simulink model "VehicleSignals"  (R2024a)
settings: Solver=FixedStepDiscrete  StartTime=0.0  StopTime=VSG_Stop_Time  FixedStep=VSG_Step_Size  RelTol=1e-3  EnableMultiTasking=on
undefined symbols (not defined in the file): GEAR_FAILSAFE, Gear_T, RadarStatus_T, SignalStatus_T, STEER_FAILSAFE_DEG, STEER_RAW_MAX, STEER_RAW_MIN, STEER_RESOLUTION_DEG, TurnSignal_T, VSG_RECOVERY_CNT, VSPD_FAILSAFE_KMH, VSPD_RAW_MAX, VSPD_RAW_MIN, VSPD_RESOLUTION_KMH
libraries: simulink x10
settings Model: DataDictionary=bsd.sldd  Creator=pc  LastModifiedBy=pc
settings OptimizationCC: DefaultParameterBehavior=Inlined  UseDivisionForNetSlopeComputation=on  DefaultUnderspecifiedDataType=single  EnhancedBackFolding=on  PassReuseOutputArgsAs=Individual arguments  ZeroExternalMemoryAtStartup=off  ZeroInternalMemoryAtStartup=off  OptimizeBlockOrder=speed  DifferentSizesBufferReuse=on  OptimizationCustomize=off  EfficientTunableParamExpr=on
settings DebuggingCC: ParameterTunabilityLossMsg=error
settings SFSimCC: MATLABDynamicMemAlloc=off
settings RTWCC: Description=AUTOSAR  SystemTargetFile=autosar.tlc  GenCodeOnly=on  TemplateMakefile=ert_default_tmf  DataTypeReplacement=CDataTypesFixedWidth
settings CodeAppCC: ForceParamTrailComments=on  IgnoreCustomStorageClasses=off  OperatorAnnotations=on  SimulinkDataObjDesc=on  SFDataObjDesc=on  InsertBlockDesc=on
settings STFCustomTargetCC: MultiwordLength=256  ParMdlRefBuildCompliant=on  CompOptLevelCompliant=on  IncludeMdlTerminateFcn=off  CombineOutputUpdateFcns=on  SuppressErrorStatus=on  ERTCustomFileBanners=on  SupportNonFinite=off  SupportComplex=off  SupportContinuousTime=off  SupportNonInlinedSFcns=off  RemoveResetFunc=on  MATLABClassNameForMDSCustomization=Simulink.SoftwareTarget.ERTCustomization  AutosarCompliant=on  GRTInterface=off  LookupTableObjectStructAxisOrder=2,1,3,4,...  LUTObjectStructOrderEvenSpacing=Size,Table,Breakpoints  SystemTargetFile=autosar.tlc
settings ERTTargetCC: TargetLangStandard=C99 (ISO)  ConcurrentExecutionCompliant=off  IncludeMdlTerminateFcn=off  SuppressErrorStatus=on  SupportNonFinite=off  SupportComplex=off  ModelStepFunctionPrototypeControlCompliant=off  CPPClassGenCompliant=off  AutosarCompliant=on  LookupTableObjectStructAxisOrder=2,1,3,4,...  LUTObjectStructOrderEvenSpacing=Size,Table,Breakpoints  InlinedParameterPlacement=NonHierarchical  ERTCustomFileTemplate=example_file_process.tlc  BooleanTrueId=TRUE  BooleanFalseId=FALSE

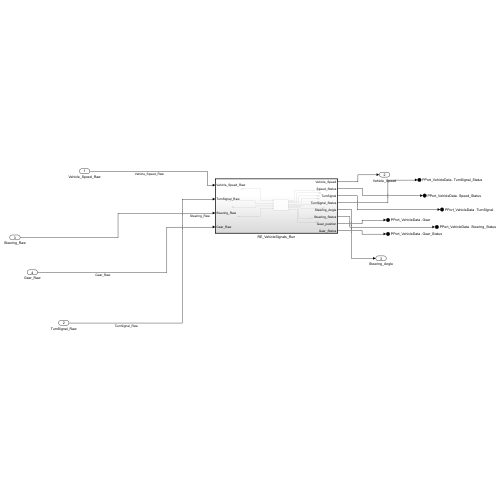
[thumbnail: Simulink's stored preview of the top-level diagram]
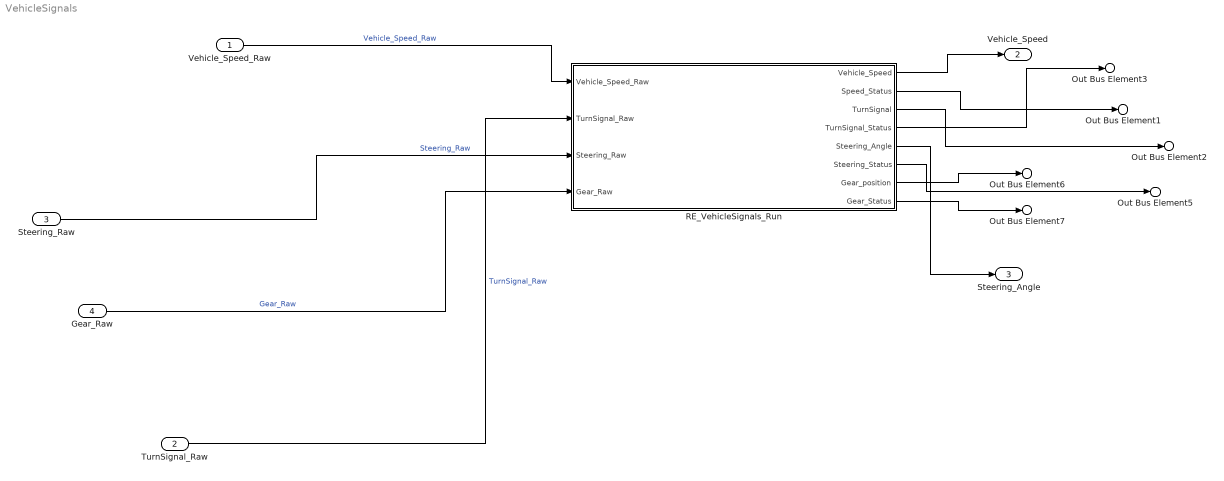
== system VehicleSignals ==
  Vehicle_Speed_Raw : Inport  OutDataTypeStr=Speed_Raw_T
  TurnSignal_Raw : Inport  Port=2  OutDataTypeStr=TurnSignal_Raw_T
  Steering_Raw : Inport  Port=3  OutDataTypeStr=Steering_Raw_T
  Gear_Raw : Inport  Port=4  OutDataTypeStr=Gear_Raw_T
  RE_VehicleSignals_Run : Subsystem  TreatAsAtomicUnit=on
  Out Bus Element5 : Outport  PortName=PPort_VehicleData  Element=Steering_Status
  Out Bus Element7 : Outport  PortName=PPort_VehicleData  Element=Gear_Status
  Out Bus Element6 : Outport  PortName=PPort_VehicleData  Element=Gear
  Out Bus Element3 : Outport  PortName=PPort_VehicleData  Element=TurnSignal_Status
  Out Bus Element2 : Outport  PortName=PPort_VehicleData  Element=TurnSignal
  Out Bus Element1 : Outport  PortName=PPort_VehicleData  Element=Speed_Status
  Vehicle_Speed : Outport  Port=2  OutDataTypeStr=Vehicle_Speed_T
  Steering_Angle : Outport  Port=3  OutDataTypeStr=Steering_Angle_T
  wires:
  RE_VehicleSignals_Run/1(Vehicle_Speed) -> Vehicle_Speed/1
  RE_VehicleSignals_Run/4(TurnSignal_Status) -> Out Bus Element3/1
  RE_VehicleSignals_Run/2(Speed_Status) -> Out Bus Element1/1
  RE_VehicleSignals_Run/5(Steering_Angle) -> Steering_Angle/1
  RE_VehicleSignals_Run/3(TurnSignal) -> Out Bus Element2/1
  RE_VehicleSignals_Run/7(Gear_position) -> Out Bus Element6/1
  RE_VehicleSignals_Run/8(Gear_Status) -> Out Bus Element7/1
  RE_VehicleSignals_Run/6(Steering_Status) -> Out Bus Element5/1
  Gear_Raw/1 -> RE_VehicleSignals_Run/4(Gear_Raw)  "Gear_Raw"
  TurnSignal_Raw/1 -> RE_VehicleSignals_Run/2(TurnSignal_Raw)  "TurnSignal_Raw"
  Vehicle_Speed_Raw/1 -> RE_VehicleSignals_Run/1(Vehicle_Speed_Raw)  "Vehicle_Speed_Raw"
  Steering_Raw/1 -> RE_VehicleSignals_Run/3(Steering_Raw)  "Steering_Raw"

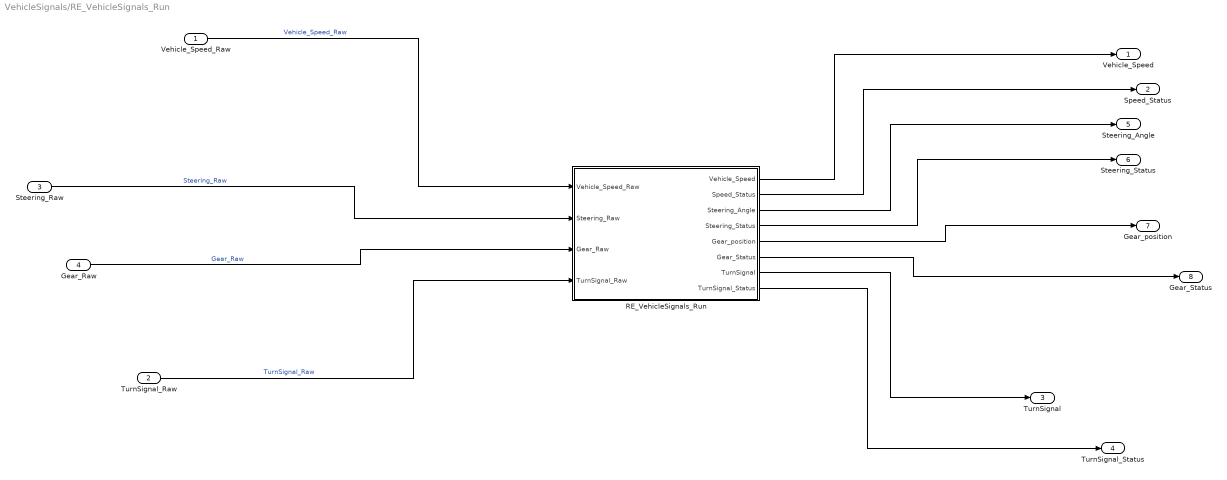
== system VehicleSignals/RE_VehicleSignals_Run ==
  Vehicle_Speed_Raw : Inport  OutDataTypeStr=Speed_Raw_T
  TurnSignal_Raw : Inport  Port=2  OutDataTypeStr=TurnSignal_Raw_T
  Steering_Raw : Inport  Port=3  OutDataTypeStr=Steering_Raw_T
  Gear_Raw : Inport  Port=4  OutDataTypeStr=Gear_Raw_T
  RE_VehicleSignals_Run : Subsystem
  Vehicle_Speed : Outport  OutDataTypeStr=Vehicle_Speed_T
  Speed_Status : Outport  Port=2  OutDataTypeStr=Enum: SignalStatus_T
  TurnSignal : Outport  Port=3  OutDataTypeStr=Enum: TurnSignal_T
  TurnSignal_Status : Outport  Port=4  OutDataTypeStr=Enum: SignalStatus_T
  Steering_Angle : Outport  Port=5  OutDataTypeStr=Steering_Angle_T
  Steering_Status : Outport  Port=6  OutDataTypeStr=Enum: SignalStatus_T
  Gear_position : Outport  Port=7  OutDataTypeStr=Enum: Gear_T
  Gear_Status : Outport  Port=8  OutDataTypeStr=Enum: SignalStatus_T
  wires:
  Vehicle_Speed_Raw/1 -> RE_VehicleSignals_Run/1(Vehicle_Speed_Raw)  "Vehicle_Speed_Raw"
  Steering_Raw/1 -> RE_VehicleSignals_Run/2(Steering_Raw)  "Steering_Raw"
  Gear_Raw/1 -> RE_VehicleSignals_Run/3(Gear_Raw)  "Gear_Raw"
  TurnSignal_Raw/1 -> RE_VehicleSignals_Run/4(TurnSignal_Raw)  "TurnSignal_Raw"
  RE_VehicleSignals_Run/1(Vehicle_Speed) -> Vehicle_Speed/1
  RE_VehicleSignals_Run/2(Speed_Status) -> Speed_Status/1
  RE_VehicleSignals_Run/3(Steering_Angle) -> Steering_Angle/1
  RE_VehicleSignals_Run/4(Steering_Status) -> Steering_Status/1
  RE_VehicleSignals_Run/5(Gear_position) -> Gear_position/1
  RE_VehicleSignals_Run/6(Gear_Status) -> Gear_Status/1
  RE_VehicleSignals_Run/7(TurnSignal) -> TurnSignal/1
  RE_VehicleSignals_Run/8(TurnSignal_Status) -> TurnSignal_Status/1

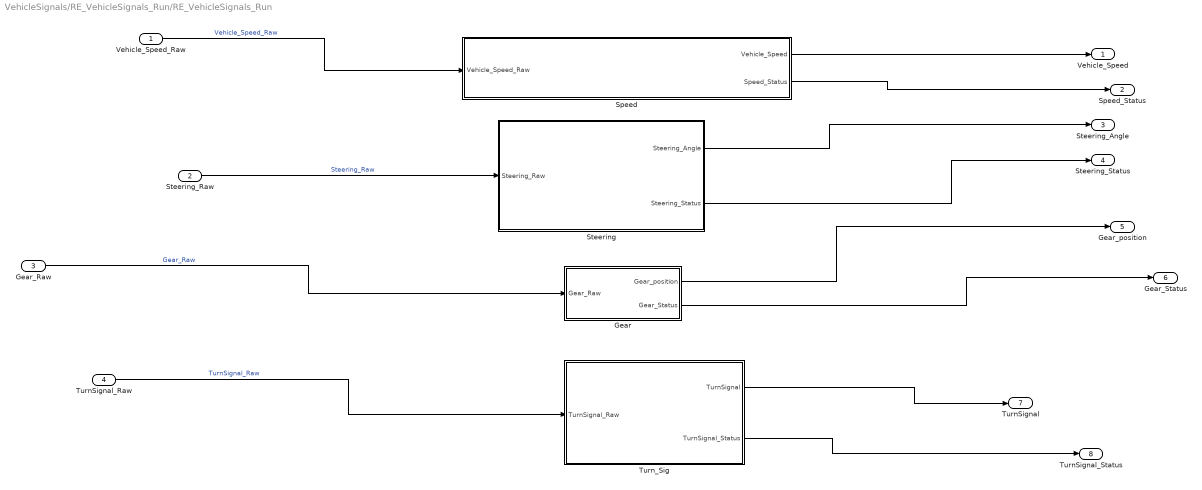
== system VehicleSignals/RE_VehicleSignals_Run/RE_VehicleSignals_Run ==
  Vehicle_Speed_Raw : Inport  OutDataTypeStr=Speed_Raw_T
  Steering_Raw : Inport  Port=2  OutDataTypeStr=Steering_Raw_T
  Gear_Raw : Inport  Port=3  OutDataTypeStr=ValueType: Gear_Raw
  TurnSignal_Raw : Inport  Port=4  OutDataTypeStr=ValueType: Raw_turn_sig
  Gear : Subsystem
  Speed : Subsystem
  Steering : Subsystem
  Turn_Sig : Subsystem
  Vehicle_Speed : Outport  OutDataTypeStr=ValueType: Vehicle_Speed
  Speed_Status : Outport  Port=2  OutDataTypeStr=Enum: SignalStatus_T
  Steering_Angle : Outport  Port=3  OutDataTypeStr=ValueType: Steering_Angle
  Steering_Status : Outport  Port=4  OutDataTypeStr=Enum: SignalStatus_T
  Gear_position : Outport  Port=5  OutDataTypeStr=Enum: Gear_T
  Gear_Status : Outport  Port=6  OutDataTypeStr=Enum: SignalStatus_T
  TurnSignal : Outport  Port=7  OutDataTypeStr=Enum: TurnSignal_T
  TurnSignal_Status : Outport  Port=8  OutDataTypeStr=Enum: SignalStatus_T
  wires:
  Vehicle_Speed_Raw/1 -> Speed/1(Vehicle_Speed_Raw)  "Vehicle_Speed_Raw"
  Steering/1(Steering_Angle) -> Steering_Angle/1
  Gear_Raw/1 -> Gear/1(Gear_Raw)  "Gear_Raw"
  Steering_Raw/1 -> Steering/1(Steering_Raw)  "Steering_Raw"
  Turn_Sig/2(TurnSignal_Status) -> TurnSignal_Status/1
  TurnSignal_Raw/1 -> Turn_Sig/1(TurnSignal_Raw)  "TurnSignal_Raw"
  Turn_Sig/1(TurnSignal) -> TurnSignal/1
  Steering/2(Steering_Status) -> Steering_Status/1
  Speed/1(Vehicle_Speed) -> Vehicle_Speed/1
  Speed/2(Speed_Status) -> Speed_Status/1
  Gear/1(Gear_position) -> Gear_position/1
  Gear/2(Gear_Status) -> Gear_Status/1

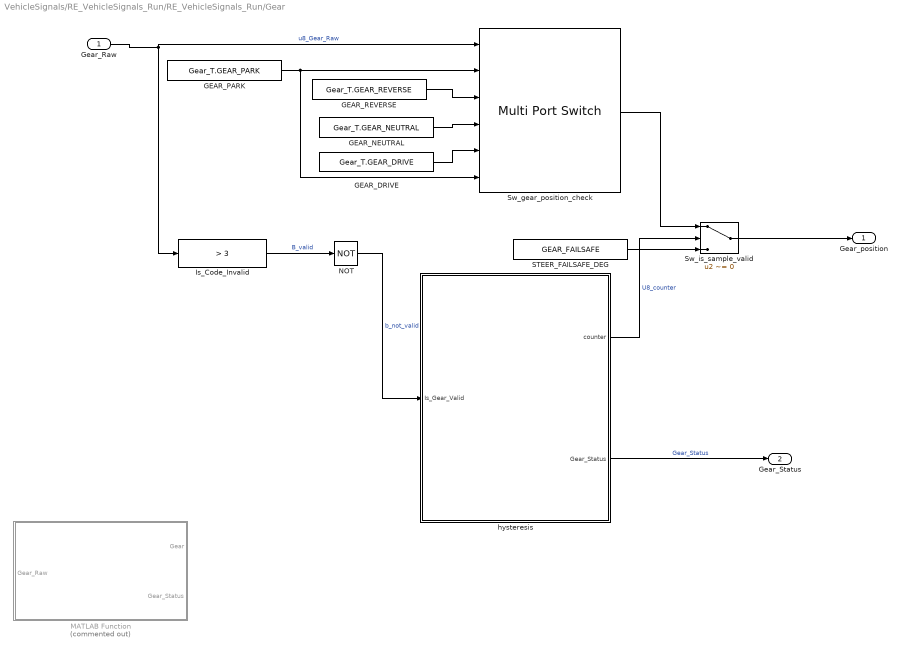
== system VehicleSignals/RE_VehicleSignals_Run/RE_VehicleSignals_Run/Gear ==
  Gear_Raw : Inport  OutDataTypeStr=ValueType: Gear_Raw
  GEAR_DRIVE : Constant  Value=Gear_T.GEAR_DRIVE  OutDataTypeStr=Enum: Gear_T
  GEAR_NEUTRAL : Constant  Value=Gear_T.GEAR_NEUTRAL  OutDataTypeStr=Enum: Gear_T
  GEAR_PARK : Constant  Value=Gear_T.GEAR_PARK  OutDataTypeStr=Enum: Gear_T
  GEAR_REVERSE : Constant  Value=Gear_T.GEAR_REVERSE  OutDataTypeStr=Enum: Gear_T
  Is_Code_Invalid : simulink/Logic and Bit Operations/Compare To Constant  relop=>  const=3  OutDataTypeStr=boolean
  MATLAB Function : MATLAB Function  Commented=on  TreatAsAtomicUnit=on
  NOT : Logic  Operator=NOT  AllPortsSameDT=off  OutDataTypeStr=boolean
  STEER_FAILSAFE_DEG : Constant  Value=GEAR_FAILSAFE  OutDataTypeStr=Enum: Gear_T
  Sw_gear_position_check : MultiPortSwitch  DataPortOrder=Specify indices  Inputs=5  DataPortIndices={0,1,2,3}  DataPortForDefault=Additional data port  DiagnosticForDefault=None  SaturateOnIntegerOverflow=off  InputSameDT=off
  Sw_is_sample_valid : Switch  Criteria=u2 ~= 0  OutDataTypeStr=Enum: Gear_T  SaturateOnIntegerOverflow=off  InputSameDT=off
  hysteresis : Subsystem
  Gear_position : Outport  OutDataTypeStr=Enum: Gear_T
  Gear_Status : Outport  Port=2  OutDataTypeStr=Enum: SignalStatus_T
  wires:
  Sw_is_sample_valid/1 -> Gear_position/1
  STEER_FAILSAFE_DEG/1 -> Sw_is_sample_valid/3
  Gear_Raw/1 -> Is_Code_Invalid/1, Sw_gear_position_check/1  "u8_Gear_Raw"
  NOT/1 -> hysteresis/1(Is_Gear_Valid)  "b_not_valid"
  hysteresis/2(Gear_Status) -> Gear_Status/1  "Gear_Status"
  hysteresis/1(counter) -> Sw_is_sample_valid/2  "U8_counter"
  Is_Code_Invalid/1 -> NOT/1  "B_valid"
  GEAR_REVERSE/1 -> Sw_gear_position_check/3
  GEAR_PARK/1 -> Sw_gear_position_check/2, Sw_gear_position_check/6
  GEAR_NEUTRAL/1 -> Sw_gear_position_check/4
  GEAR_DRIVE/1 -> Sw_gear_position_check/5
  Sw_gear_position_check/1 -> Sw_is_sample_valid/1

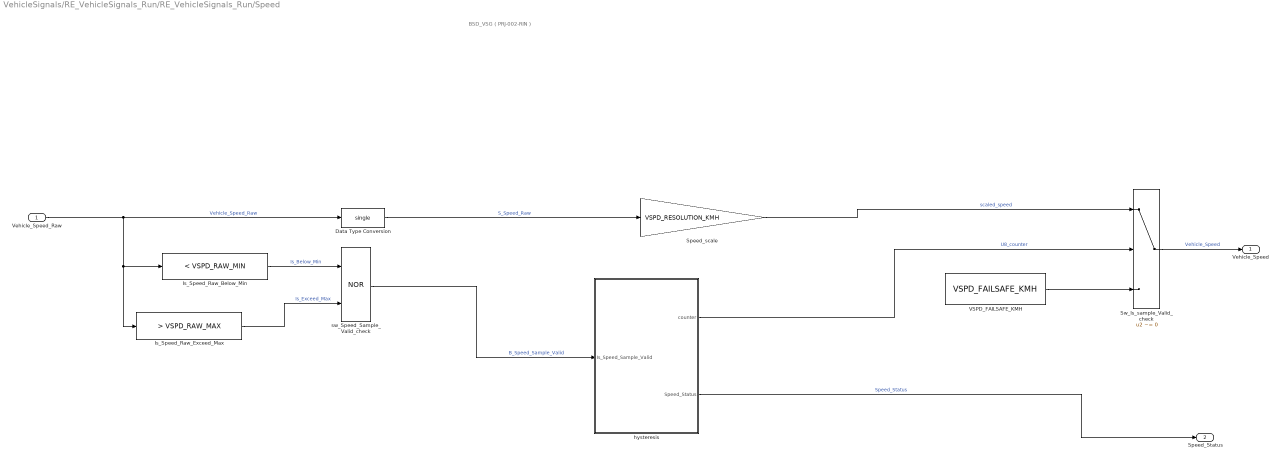
== system VehicleSignals/RE_VehicleSignals_Run/RE_VehicleSignals_Run/Speed ==
  note: BSD_VSG ( PRJ-002-RIN )
  Vehicle_Speed_Raw : Inport  OutDataTypeStr=ValueType: Vehicle_Speed_Raw
  Data Type Conversion : DataTypeConversion  OutDataTypeStr=single  SaturateOnIntegerOverflow=off  RndMeth=Floor
  Is_Speed_Raw_Below_Min : simulink/Logic and Bit Operations/Compare To Constant  relop=<  const=VSPD_RAW_MIN  OutDataTypeStr=uint8
  Is_Speed_Raw_Exceed_Max : simulink/Logic and Bit Operations/Compare To Constant  relop=>  const=VSPD_RAW_MAX  OutDataTypeStr=uint8
  Speed_scale : Gain  Gain=VSPD_RESOLUTION_KMH  OutDataTypeStr=single
  Sw_Is_sample_Valid_check : Switch  Criteria=u2 ~= 0  OutDataTypeStr=single  SaturateOnIntegerOverflow=off  InputSameDT=off
  VSPD_FAILSAFE_KMH : Constant  Value=VSPD_FAILSAFE_KMH  OutDataTypeStr=ValueType: Vehicle_Speed
  hysteresis : Subsystem
  sw_Speed_Sample_Valid_check : Logic  Operator=NOR  AllPortsSameDT=off  OutDataTypeStr=boolean
  Vehicle_Speed : Outport  OutDataTypeStr=ValueType: Vehicle_Speed
  Speed_Status : Outport  Port=2  OutDataTypeStr=Enum: SignalStatus_T
  wires:
  Is_Speed_Raw_Exceed_Max/1 -> sw_Speed_Sample_Valid_check/2  "Is_Exceed_Max"
  Is_Speed_Raw_Below_Min/1 -> sw_Speed_Sample_Valid_check/1  "Is_Below_Min"
  Speed_scale/1 -> Sw_Is_sample_Valid_check/1  "scaled_speed"
  Data Type Conversion/1 -> Speed_scale/1  "S_Speed_Raw"
  Sw_Is_sample_Valid_check/1 -> Vehicle_Speed/1  "Vehicle_Speed"
  VSPD_FAILSAFE_KMH/1 -> Sw_Is_sample_Valid_check/3
  Vehicle_Speed_Raw/1 -> Is_Speed_Raw_Exceed_Max/1, Is_Speed_Raw_Below_Min/1, Data Type Conversion/1  "Vehicle_Speed_Raw"
  sw_Speed_Sample_Valid_check/1 -> hysteresis/1(Is_Speed_Sample_Valid)  "B_Speed_Sample_Valid"
  hysteresis/1(counter) -> Sw_Is_sample_Valid_check/2  "U8_counter"
  hysteresis/2(Speed_Status) -> Speed_Status/1  "Speed_Status"

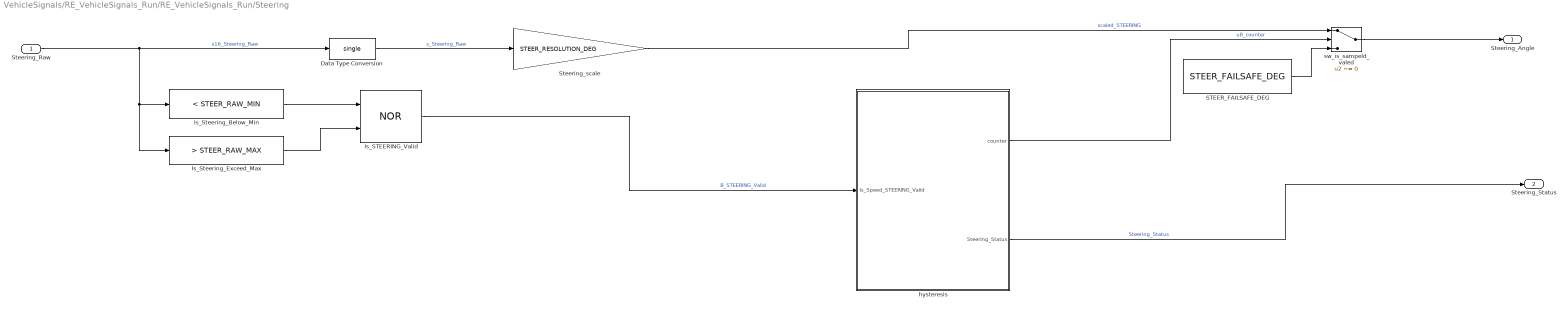
== system VehicleSignals/RE_VehicleSignals_Run/RE_VehicleSignals_Run/Steering ==
  Steering_Raw : Inport  OutDataTypeStr=Steering_Raw_T
  Data Type Conversion : DataTypeConversion  OutDataTypeStr=single  SaturateOnIntegerOverflow=off  RndMeth=Floor
  "Is_STEERING_Valid " : Logic  Operator=NOR  AllPortsSameDT=off  OutDataTypeStr=boolean
  Is_Steering_Below_Min : simulink/Logic and Bit Operations/Compare To Constant  relop=<  const=STEER_RAW_MIN  OutDataTypeStr=uint8
  Is_Steering_Exceed_Max : simulink/Logic and Bit Operations/Compare To Constant  relop=>  const=STEER_RAW_MAX  OutDataTypeStr=uint8
  STEER_FAILSAFE_DEG : Constant  Value=STEER_FAILSAFE_DEG  OutDataTypeStr=ValueType: Vehicle_Speed
  Steering_scale : Gain  Gain=STEER_RESOLUTION_DEG  OutDataTypeStr=single
  hysteresis : Subsystem
  sw_is_sampeld_valed : Switch  Criteria=u2 ~= 0  OutDataTypeStr=single  SaturateOnIntegerOverflow=off  InputSameDT=off
  Steering_Angle : Outport  OutDataTypeStr=ValueType: Steering_Angle
  Steering_Status : Outport  Port=2  OutDataTypeStr=Enum: SignalStatus_T
  wires:
  sw_is_sampeld_valed/1 -> Steering_Angle/1
  STEER_FAILSAFE_DEG/1 -> sw_is_sampeld_valed/3
  Steering_scale/1 -> sw_is_sampeld_valed/1  "scaled_STEERING"
  Steering_Raw/1 -> Is_Steering_Exceed_Max/1, Is_Steering_Below_Min/1, Data Type Conversion/1  "s16_Steering_Raw"
  Is_Steering_Exceed_Max/1 -> "Is_STEERING_Valid "/2
  Is_Steering_Below_Min/1 -> "Is_STEERING_Valid "/1
  "Is_STEERING_Valid "/1 -> hysteresis/1(Is_Speed_STEERING_Valid)  "B_STEERING_Valid"
  hysteresis/1(counter) -> sw_is_sampeld_valed/2  "u8_counter"
  hysteresis/2(Steering_Status) -> Steering_Status/1  "Steering_Status"
  Data Type Conversion/1 -> Steering_scale/1  "s_Steering_Raw"

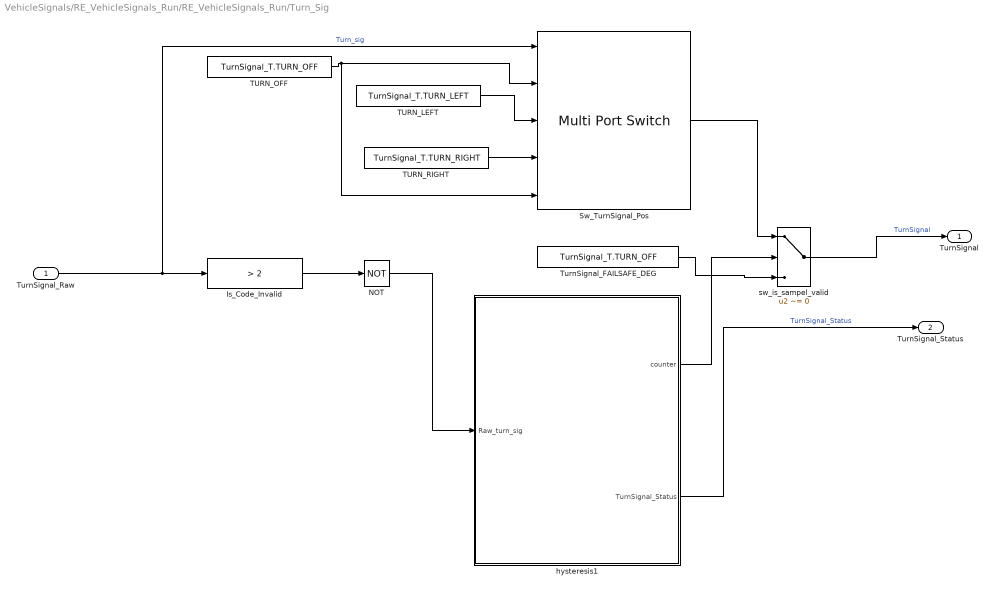
== system VehicleSignals/RE_VehicleSignals_Run/RE_VehicleSignals_Run/Turn_Sig ==
  TurnSignal_Raw : Inport
  Is_Code_Invalid : simulink/Logic and Bit Operations/Compare To Constant  relop=>  const=2  OutDataTypeStr=boolean
  NOT : Logic  Operator=NOT  AllPortsSameDT=off  OutDataTypeStr=boolean
  Sw_TurnSignal_Pos : MultiPortSwitch  DataPortOrder=Specify indices  Inputs=5  DataPortIndices={0,1,2}  DataPortForDefault=Additional data port  DiagnosticForDefault=None  SaturateOnIntegerOverflow=off  InputSameDT=off
  TURN_LEFT : Constant  Value=TurnSignal_T.TURN_LEFT  OutDataTypeStr=Enum: TurnSignal_T
  TURN_OFF : Constant  Value=TurnSignal_T.TURN_OFF  OutDataTypeStr=Enum: TurnSignal_T
  TURN_RIGHT : Constant  Value=TurnSignal_T.TURN_RIGHT  OutDataTypeStr=Enum: TurnSignal_T
  TurnSignal_FAILSAFE_DEG : Constant  Value=TurnSignal_T.TURN_OFF  OutDataTypeStr=Enum: TurnSignal_T
  hysteresis1 : Subsystem
  sw_is_sampel_valid : Switch  Criteria=u2 ~= 0  OutDataTypeStr=Enum: TurnSignal_T  SaturateOnIntegerOverflow=off  InputSameDT=off
  TurnSignal : Outport  OutDataTypeStr=Enum: TurnSignal_T
  TurnSignal_Status : Outport  Port=2  OutDataTypeStr=Enum: SignalStatus_T
  wires:
  TurnSignal_Raw/1 -> Sw_TurnSignal_Pos/1, Is_Code_Invalid/1  "Turn_sig"
  Sw_TurnSignal_Pos/1 -> sw_is_sampel_valid/1
  NOT/1 -> hysteresis1/1(Raw_turn_sig)
  TurnSignal_FAILSAFE_DEG/1 -> sw_is_sampel_valid/3
  Is_Code_Invalid/1 -> NOT/1
  hysteresis1/2(TurnSignal_Status) -> TurnSignal_Status/1  "TurnSignal_Status"
  TURN_RIGHT/1 -> Sw_TurnSignal_Pos/4
  hysteresis1/1(counter) -> sw_is_sampel_valid/2
  TURN_LEFT/1 -> Sw_TurnSignal_Pos/3
  TURN_OFF/1 -> Sw_TurnSignal_Pos/5, Sw_TurnSignal_Pos/2
  sw_is_sampel_valid/1 -> TurnSignal/1  "TurnSignal"

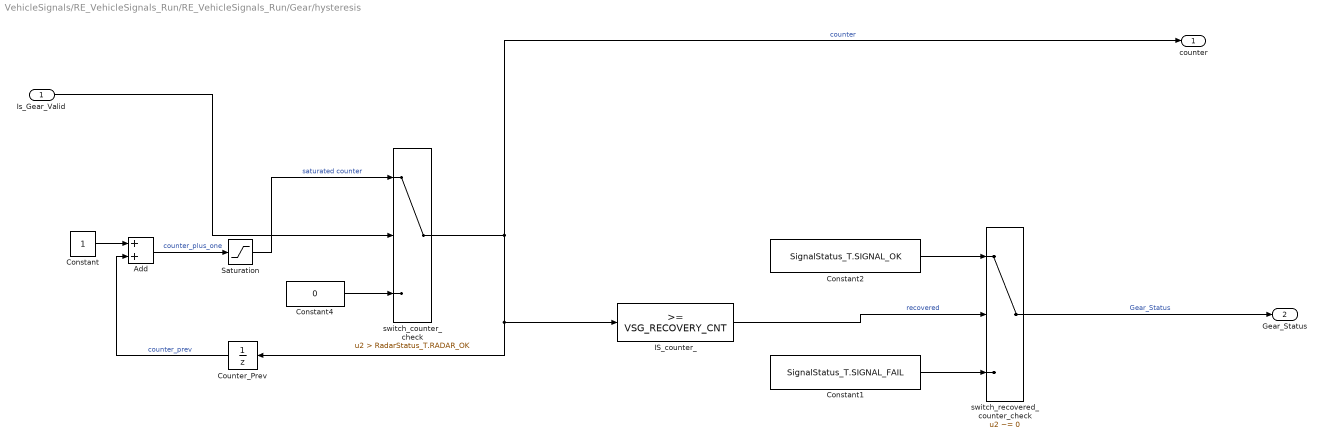
== system VehicleSignals/RE_VehicleSignals_Run/RE_VehicleSignals_Run/Gear/hysteresis ==
  Is_Gear_Valid : Inport
  Add : Sum  OutDataTypeStr=uint8
  Constant : Constant  OutDataTypeStr=uint8
  Constant1 : Constant  Value=SignalStatus_T.SIGNAL_FAIL  OutDataTypeStr=Enum: SignalStatus_T
  Constant2 : Constant  Value=SignalStatus_T.SIGNAL_OK  OutDataTypeStr=Enum: SignalStatus_T
  Constant4 : Constant  Value=0  OutDataTypeStr=uint8
  Counter_Prev : UnitDelay  SampleTime=-1  HasFrameUpgradeWarning=on
  IS_counter_ : simulink/Logic and Bit Operations/Compare To Constant  relop=>=  const=VSG_RECOVERY_CNT  OutDataTypeStr=boolean
  Saturation : Saturate  UpperLimit=3  LowerLimit=0  OutDataTypeStr=uint8
  switch_counter_check : Switch  Criteria=u2 > Threshold  Threshold=RadarStatus_T.RADAR_OK  OutDataTypeStr=uint8  SaturateOnIntegerOverflow=off  InputSameDT=off
  switch_recovered_counter_check : Switch  Criteria=u2 ~= 0  OutDataTypeStr=Enum: SignalStatus_T  SaturateOnIntegerOverflow=off  InputSameDT=off
  counter : Outport  OutDataTypeStr=uint8
  Gear_Status : Outport  Port=2
  wires:
  Constant4/1 -> switch_counter_check/3
  switch_counter_check/1 -> counter/1, Counter_Prev/1, IS_counter_/1  "counter"
  Add/1 -> Saturation/1  "counter_plus_one"
  Constant2/1 -> switch_recovered_counter_check/1
  Constant1/1 -> switch_recovered_counter_check/3
  Counter_Prev/1 -> Add/2  "counter_prev"
  Constant/1 -> Add/1
  IS_counter_/1 -> switch_recovered_counter_check/2  "recovered"
  Saturation/1 -> switch_counter_check/1  "saturated counter"
  Is_Gear_Valid/1 -> switch_counter_check/2
  switch_recovered_counter_check/1 -> Gear_Status/1  "Gear_Status"

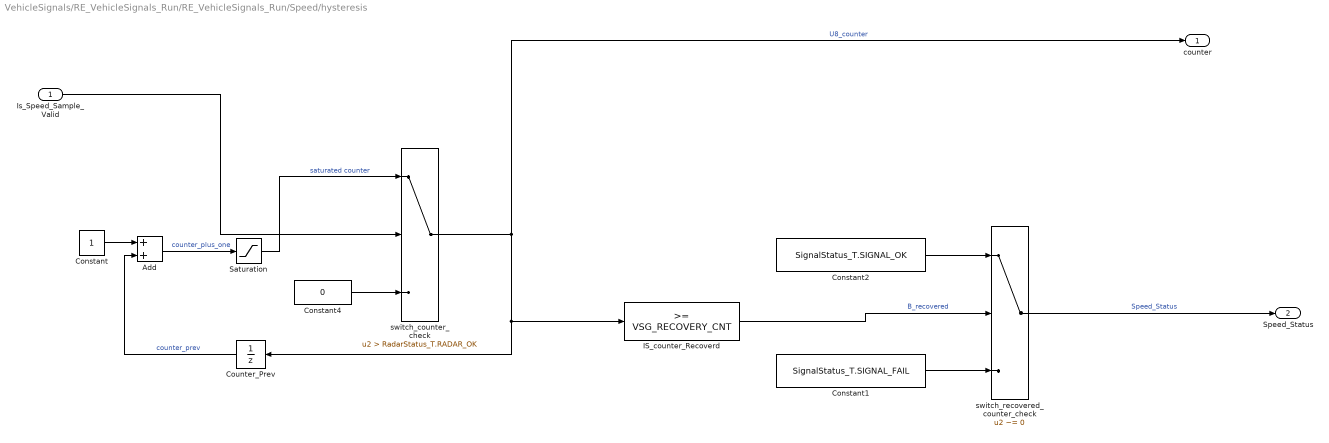
== system VehicleSignals/RE_VehicleSignals_Run/RE_VehicleSignals_Run/Speed/hysteresis ==
  Is_Speed_Sample_Valid : Inport
  Add : Sum  OutDataTypeStr=uint8
  Constant : Constant  OutDataTypeStr=uint8
  Constant1 : Constant  Value=SignalStatus_T.SIGNAL_FAIL  OutDataTypeStr=Enum: SignalStatus_T
  Constant2 : Constant  Value=SignalStatus_T.SIGNAL_OK  OutDataTypeStr=Enum: SignalStatus_T
  Constant4 : Constant  Value=0
  Counter_Prev : UnitDelay  SampleTime=-1  HasFrameUpgradeWarning=on
  IS_counter_Recoverd : simulink/Logic and Bit Operations/Compare To Constant  relop=>=  const=VSG_RECOVERY_CNT  OutDataTypeStr=boolean
  Saturation : Saturate  UpperLimit=3  LowerLimit=0  OutDataTypeStr=uint8
  switch_counter_check : Switch  Criteria=u2 > Threshold  Threshold=RadarStatus_T.RADAR_OK  OutDataTypeStr=uint8  SaturateOnIntegerOverflow=off  InputSameDT=off
  switch_recovered_counter_check : Switch  Criteria=u2 ~= 0  OutDataTypeStr=Enum: SignalStatus_T  SaturateOnIntegerOverflow=off  InputSameDT=off
  counter : Outport
  Speed_Status : Outport  Port=2
  wires:
  Constant4/1 -> switch_counter_check/3
  switch_counter_check/1 -> counter/1, Counter_Prev/1, IS_counter_Recoverd/1  "U8_counter"
  Add/1 -> Saturation/1  "counter_plus_one"
  Constant2/1 -> switch_recovered_counter_check/1
  Constant1/1 -> switch_recovered_counter_check/3
  Counter_Prev/1 -> Add/2  "counter_prev"
  Constant/1 -> Add/1
  IS_counter_Recoverd/1 -> switch_recovered_counter_check/2  "B_recovered"
  Saturation/1 -> switch_counter_check/1  "saturated counter"
  Is_Speed_Sample_Valid/1 -> switch_counter_check/2
  switch_recovered_counter_check/1 -> Speed_Status/1  "Speed_Status"

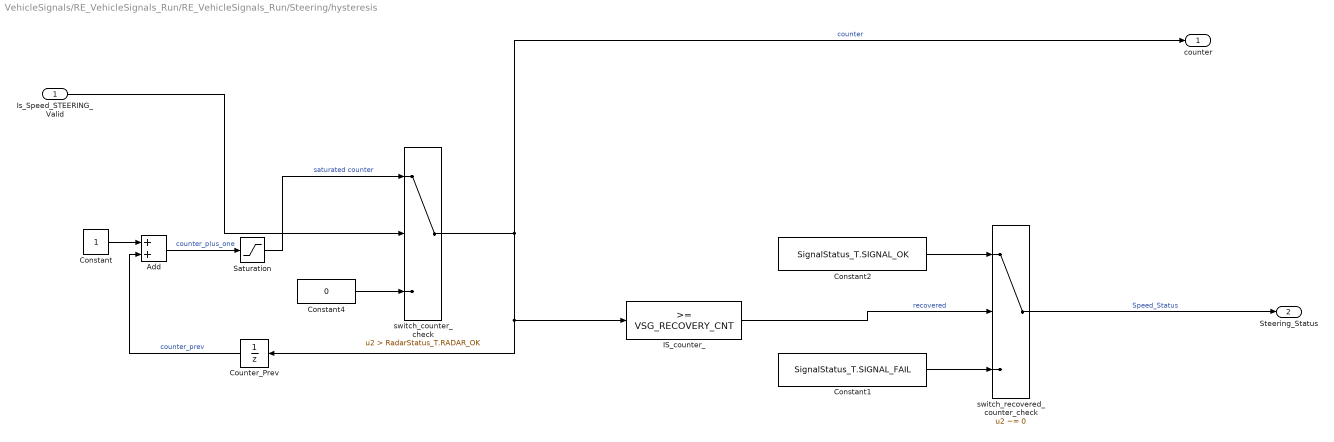
== system VehicleSignals/RE_VehicleSignals_Run/RE_VehicleSignals_Run/Steering/hysteresis ==
  Is_Speed_STEERING_Valid : Inport
  Add : Sum  OutDataTypeStr=uint8
  Constant : Constant  OutDataTypeStr=uint8
  Constant1 : Constant  Value=SignalStatus_T.SIGNAL_FAIL  OutDataTypeStr=Enum: SignalStatus_T
  Constant2 : Constant  Value=SignalStatus_T.SIGNAL_OK  OutDataTypeStr=Enum: SignalStatus_T
  Constant4 : Constant  Value=0
  Counter_Prev : UnitDelay  SampleTime=-1  HasFrameUpgradeWarning=on
  IS_counter_ : simulink/Logic and Bit Operations/Compare To Constant  relop=>=  const=VSG_RECOVERY_CNT  OutDataTypeStr=boolean
  Saturation : Saturate  UpperLimit=3  LowerLimit=0  OutDataTypeStr=uint8
  switch_counter_check : Switch  Criteria=u2 > Threshold  Threshold=RadarStatus_T.RADAR_OK  OutDataTypeStr=uint8  SaturateOnIntegerOverflow=off  InputSameDT=off
  switch_recovered_counter_check : Switch  Criteria=u2 ~= 0  OutDataTypeStr=Enum: SignalStatus_T  SaturateOnIntegerOverflow=off  InputSameDT=off
  counter : Outport
  Steering_Status : Outport  Port=2
  wires:
  Constant4/1 -> switch_counter_check/3
  switch_counter_check/1 -> counter/1, Counter_Prev/1, IS_counter_/1  "counter"
  Add/1 -> Saturation/1  "counter_plus_one"
  Constant2/1 -> switch_recovered_counter_check/1
  Constant1/1 -> switch_recovered_counter_check/3
  Counter_Prev/1 -> Add/2  "counter_prev"
  Constant/1 -> Add/1
  IS_counter_/1 -> switch_recovered_counter_check/2  "recovered"
  Saturation/1 -> switch_counter_check/1  "saturated counter"
  Is_Speed_STEERING_Valid/1 -> switch_counter_check/2
  switch_recovered_counter_check/1 -> Steering_Status/1  "Speed_Status"

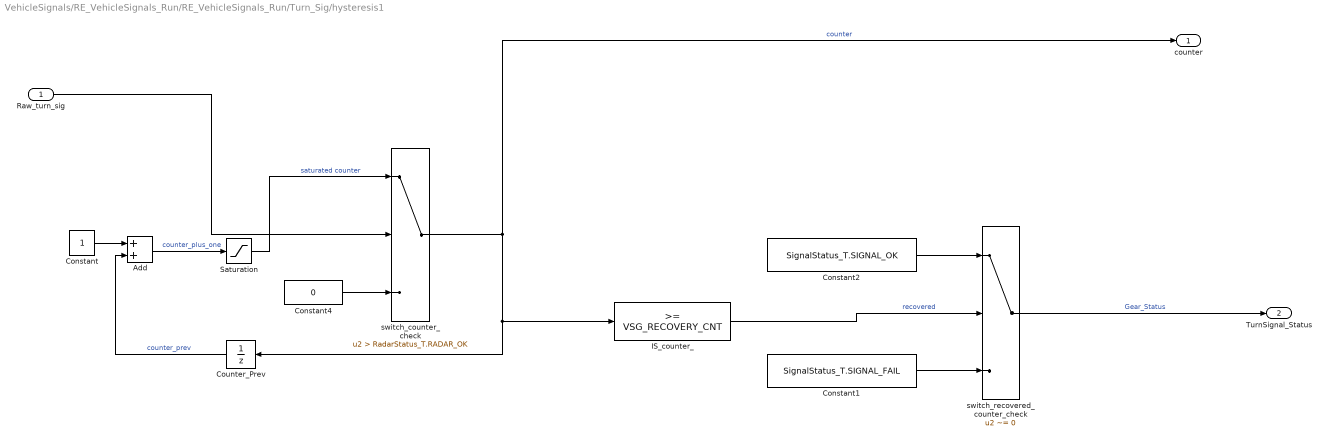
== system VehicleSignals/RE_VehicleSignals_Run/RE_VehicleSignals_Run/Turn_Sig/hysteresis1 ==
  Raw_turn_sig : Inport
  Add : Sum  OutDataTypeStr=uint8
  Constant : Constant  OutDataTypeStr=uint8
  Constant1 : Constant  Value=SignalStatus_T.SIGNAL_FAIL  OutDataTypeStr=Enum: SignalStatus_T
  Constant2 : Constant  Value=SignalStatus_T.SIGNAL_OK  OutDataTypeStr=Enum: SignalStatus_T
  Constant4 : Constant  Value=0  OutDataTypeStr=uint8
  Counter_Prev : UnitDelay  SampleTime=-1  HasFrameUpgradeWarning=on
  IS_counter_ : simulink/Logic and Bit Operations/Compare To Constant  relop=>=  const=VSG_RECOVERY_CNT  OutDataTypeStr=boolean
  Saturation : Saturate  UpperLimit=3  LowerLimit=0  OutDataTypeStr=uint8
  switch_counter_check : Switch  Criteria=u2 > Threshold  Threshold=RadarStatus_T.RADAR_OK  OutDataTypeStr=uint8  SaturateOnIntegerOverflow=off  InputSameDT=off
  switch_recovered_counter_check : Switch  Criteria=u2 ~= 0  OutDataTypeStr=Enum: SignalStatus_T  SaturateOnIntegerOverflow=off  InputSameDT=off
  counter : Outport  OutDataTypeStr=uint8
  TurnSignal_Status : Outport  Port=2
  wires:
  Constant4/1 -> switch_counter_check/3
  switch_counter_check/1 -> counter/1, Counter_Prev/1, IS_counter_/1  "counter"
  Add/1 -> Saturation/1  "counter_plus_one"
  Constant2/1 -> switch_recovered_counter_check/1
  Constant1/1 -> switch_recovered_counter_check/3
  Counter_Prev/1 -> Add/2  "counter_prev"
  Constant/1 -> Add/1
  IS_counter_/1 -> switch_recovered_counter_check/2  "recovered"
  Saturation/1 -> switch_counter_check/1  "saturated counter"
  Raw_turn_sig/1 -> switch_counter_check/2
  switch_recovered_counter_check/1 -> TurnSignal_Status/1  "Gear_Status"

== matlab function VehicleSignals/RE_VehicleSignals_Run/RE_VehicleSignals_Run/Gear/MATLAB Function ==
  data: Gear_Raw input; Gear output Enum: Gear_T; Gear_Status output Enum: SignalStatus_T
function [Gear, Gear_Status] = fcn(Gear_Raw)
    if Gear_Raw == 0
        Gear = Gear_T.GEAR_PARK;
        Gear_Status = SignalStatus_T.SIGNAL_OK;
    elseif Gear_Raw == 1
        Gear = Gear_T.GEAR_REVERSE;
        Gear_Status = SignalStatus_T.SIGNAL_OK;
    elseif Gear_Raw == 2
        Gear = Gear_T.GEAR_NEUTRAL;
        Gear_Status = SignalStatus_T.SIGNAL_OK;
    elseif Gear_Raw == 3
        Gear = Gear_T.GEAR_DRIVE;
        Gear_Status = SignalStatus_T.SIGNAL_OK;
    else
        Gear = Gear_T.GEAR_PARK;   % Fail-Safe value
        Gear_Status = SignalStatus_T.SIGNAL_FAIL;
    end
end
